simulink model "Rob_Tracking_lab"  (R2024b)
settings: Solver=FixedStepDiscrete  StartTime=0.0  StopTime=10.0  FixedStep=0.01  RelTol=1e-3  EnableMultiTasking=on
undefined symbols (not defined in the file): C_filter, DiscIntNeverNeededParam, drv, dspblkCoreblockFVToolHelper, gbox, gcbh, K_Rob_LQR, Ki, Nu, Nx, sens, T, wheel
libraries: BalRobTbx_baselib x9
settings Model: ExtModeTrigDuration=2  Creator=aboulenien  LastModifiedBy=aboulenien
settings SolverCC: AutoInsertRateTranBlk=on
settings OptimizationCC: EnhancedBackFolding=on  PassReuseOutputArgsAs=Individual arguments  ZeroExternalMemoryAtStartup=off  ZeroInternalMemoryAtStartup=off  MaxStackSize=64  OptimizeBlockOrder=speed  DifferentSizesBufferReuse=on  OptimizationCustomize=off  EfficientTunableParamExpr=on
settings DebuggingCC: ParameterTunabilityLossMsg=error
settings HardwareCC: ProdBitPerInt=16  ProdBitPerPointer=16  ProdBitPerSizeT=16  ProdBitPerPtrDiffT=16  ProdLargestAtomicFloat=None  ProdWordSize=8  ProdHWDeviceType=Atmel->AVR
settings SFSimCC: MATLABDynamicMemAlloc=off
settings RTWCC: Description=Embedded Coder  SystemTargetFile=ert.tlc  HardwareBoard=Arduino Mega 2560  TemplateMakefile=ert_default_tmf  Toolchain=Arduino AVR  BuildConfiguration=Faster Runs
settings CodeAppCC: ForceParamTrailComments=on  IgnoreCustomStorageClasses=off  OperatorAnnotations=on  SimulinkDataObjDesc=on  SFDataObjDesc=on  InsertBlockDesc=on
settings ERTTargetCC: SupportContinuousTime=on  SupportVariableSizeSignals=on  ExtModeTransport=3  ExtModeStaticAlloc=on  ExtModeAutomaticAllocSize=off  ExtModeStaticAllocSize=2048  ExtModeMexFile=ext_xcp  ExtModeIntrfLevel=Level2 - Open  InlinedParameterPlacement=Hierarchical

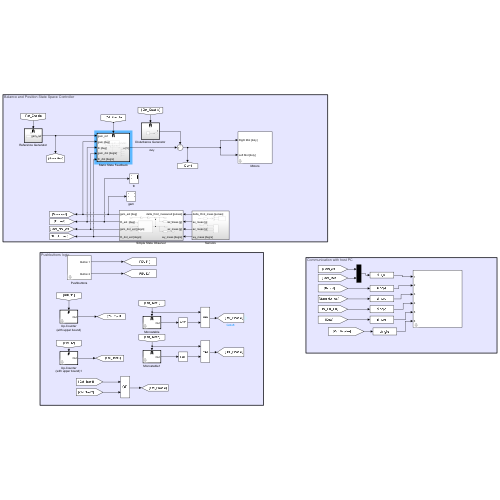
[thumbnail: Simulink's stored preview of the top-level diagram]
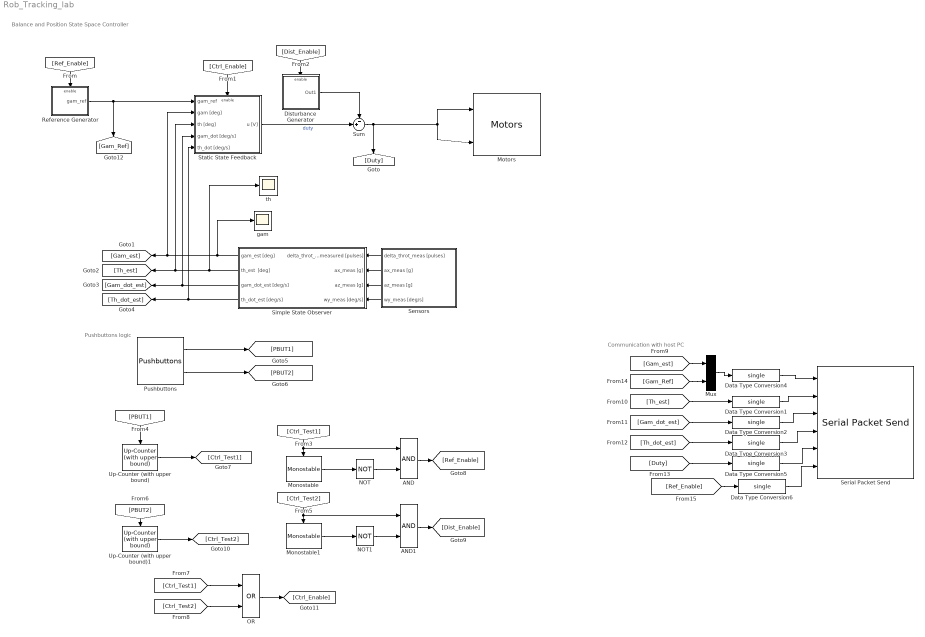
== system Rob_Tracking_lab ==
  note: Communication with host PC
  note: Balance and Position State Space Controller
  note: Pushbuttons logic
  AND : Logic  AllPortsSameDT=off  OutDataTypeStr=boolean
  AND1 : Logic  AllPortsSameDT=off  OutDataTypeStr=boolean
  Data Type Conversion{1..6} (6 alike) : DataTypeConversion  OutDataTypeStr=single  SaturateOnIntegerOverflow=off  RndMeth=Floor
  Disturbance Generator : Subsystem
  Monostable : BalRobTbx_baselib/Utilities/Monostable  Tp=5
      settings: SourceProductName=Balancing Robot Toolbox
  Monostable1 : BalRobTbx_baselib/Utilities/Monostable  Tp=1
      settings: SourceProductName=Balancing Robot Toolbox
  Motors : BalRobTbx_baselib/Outputs/Motors
      settings: SourceProductName=Balancing Robot Toolbox
  Mux : Mux  Inputs=2
  NOT : Logic  Operator=NOT  AllPortsSameDT=off  OutDataTypeStr=boolean
  NOT1 : Logic  Operator=NOT  AllPortsSameDT=off  OutDataTypeStr=boolean
  OR : Logic  Operator=OR  AllPortsSameDT=off  OutDataTypeStr=boolean
  Pushbuttons : BalRobTbx_baselib/Inputs/Pushbuttons
      settings: SourceProductName=Balancing Robot Toolbox
  Reference Generator : Subsystem
  Sensors : Subsystem
  Serial Packet Send : BalRobTbx_baselib/Communication/Serial Packet Send  serialLinkOpt=Bluetooth  baudRateOpt=38400  waitHostTxCmd=on  txStartCmd=65  txStopCmd=66  packetSpec={'2*single', 'single', 'single', 'single', 'single', 'single'}  cobsEncoded=on  nullTerminated=on  showEnablePort=off
      settings: SourceProductName=Balancing Robot Toolbox
  Simple State Observer : Subsystem
  Static State Feedback : Subsystem
  Sum : Sum  Inputs=-+|
  Up-Counter (with upper bound) : BalRobTbx_baselib/Utilities/Up-Counter (with upper bound)  CMAX=10  C0=0
      settings: SourceProductName=Balancing Robot Toolbox
  Up-Counter (with upper bound)1 : BalRobTbx_baselib/Utilities/Up-Counter (with upper bound)  CMAX=10  C0=0
      settings: SourceProductName=Balancing Robot Toolbox
  gam : Scope
  th : Scope
  wires:
  Data Type Conversion3/1 -> Serial Packet Send/4
  AND1/1 -> [Dist_Enable]
  Sensors/1(delta_throt_meas [pulses]) -> Simple State Observer/1(delta_throt_measured [pulses])
  [Ref_Enable] -> Reference Generator/Enable
  [Ctrl_Test1] -> Monostable/Enable, AND/1
  Static State Feedback/1(u [V]) -> Sum/2  "duty"
  Simple State Observer/3(gam_dot_est [deg/s]) -> Static State Feedback/4(gam_dot [deg/s]), [Gam_dot_est]
  Simple State Observer/1(gam_est [deg]) -> gam/1, Static State Feedback/2(gam [deg]), [Gam_est]
  [Ctrl_Test2] -> Monostable1/Enable, AND1/1
  [Ctrl_Test1] -> OR/1
  [Ctrl_Test2] -> OR/2
  Sensors/4(wy_meas [deg/s]) -> Simple State Observer/4(wy_meas [deg/s])
  [Ctrl_Enable] -> Static State Feedback/Enable
  Sensors/2(ax_meas [g]) -> Simple State Observer/2(ax_meas [g])
  NOT1/1 -> AND1/2
  OR/1 -> [Ctrl_Enable]
  Sensors/3(az_meas [g]) -> Simple State Observer/3(az_meas [g])
  [Dist_Enable] -> Disturbance Generator/Enable
  NOT/1 -> AND/2
  Simple State Observer/4(th_dot_est [deg/s]) -> Static State Feedback/5(th_dot [deg/s]), [Th_dot_est]
  Simple State Observer/2(th_est  [deg]) -> th/1, Static State Feedback/3(th [deg]), [Th_est]
  AND/1 -> [Ref_Enable]
  Pushbuttons/1 -> [PBUT1]
  Pushbuttons/2 -> [PBUT2]
  Data Type Conversion5/1 -> Serial Packet Send/5
  Data Type Conversion2/1 -> Serial Packet Send/3
  Data Type Conversion1/1 -> Serial Packet Send/2
  Data Type Conversion4/1 -> Serial Packet Send/1
  [Gam_est] -> Mux/1
  [Gam_Ref] -> Mux/2
  [Duty] -> Data Type Conversion5/1
  [Th_dot_est] -> Data Type Conversion3/1
  [Gam_dot_est] -> Data Type Conversion2/1
  [Th_est] -> Data Type Conversion1/1
  Mux/1 -> Data Type Conversion4/1
  Monostable1/1 -> NOT1/1
  Monostable/1 -> NOT/1
  [PBUT1] -> Up-Counter (with upper bound)/Trigger
  Up-Counter (with upper bound)/1 -> [Ctrl_Test1]
  [PBUT2] -> Up-Counter (with upper bound)1/Trigger
  Up-Counter (with upper bound)1/1 -> [Ctrl_Test2]
  [Ref_Enable] -> Data Type Conversion6/1
  Data Type Conversion6/1 -> Serial Packet Send/6
  Reference Generator/1(gam_ref) -> Static State Feedback/1(gam_ref), [Gam_Ref]
  Disturbance Generator/1(Out1) -> Sum/1
  Sum/1 -> [Duty], Motors/2, Motors/1

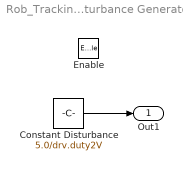
== system Rob_Tracking_lab/Disturbance Generator ==
  Enable : EnablePort  StatesWhenEnabling=reset
  Constant Disturbance : Constant  Value=5.0/drv.duty2V
  Out1 : Outport  OutputWhenDisabled=reset  InitialOutput=0
  wires:
  Constant Disturbance/1 -> Out1/1

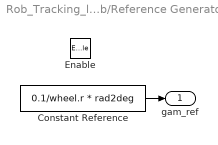
== system Rob_Tracking_lab/Reference Generator ==
  Enable : EnablePort  StatesWhenEnabling=reset
  Constant Reference : Constant  Value=0.1/wheel.r * rad2deg
  gam_ref : Outport  InitialOutput=0
  wires:
  Constant Reference/1 -> gam_ref/1

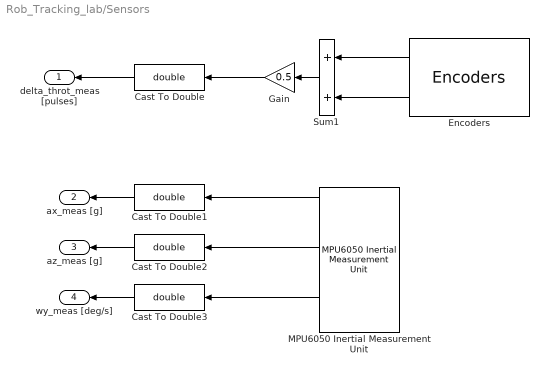
== system Rob_Tracking_lab/Sensors ==
  Cast To Double{,1..3} (4 alike) : DataTypeConversion  OutDataTypeStr=double  SaturateOnIntegerOverflow=off  RndMeth=Floor
  Encoders : BalRobTbx_baselib/Inputs/Encoders
      settings: SourceProductName=Balancing Robot Toolbox
  Gain : Gain  Gain=0.5
  MPU6050 Inertial Measurement Unit : BalRobTbx_baselib/Inputs/MPU6050 Inertial Measurement Unit
      settings: SourceProductName=Balancing Robot Toolbox
  Sum1 : Sum
  delta_throt_meas [pulses] : Outport
  ax_meas [g] : Outport  Port=2
  az_meas [g] : Outport  Port=3
  wy_meas [deg/s] : Outport  Port=4
  wires:
  Sum1/1 -> Gain/1
  Gain/1 -> Cast To Double/1
  Cast To Double/1 -> delta_throt_meas [pulses]/1
  Cast To Double3/1 -> wy_meas [deg/s]/1
  Cast To Double2/1 -> az_meas [g]/1
  Cast To Double1/1 -> ax_meas [g]/1
  Encoders/2 -> Sum1/2
  Encoders/1 -> Sum1/1
  MPU6050 Inertial Measurement Unit/1 -> Cast To Double1/1
  MPU6050 Inertial Measurement Unit/3 -> Cast To Double2/1
  MPU6050 Inertial Measurement Unit/5 -> Cast To Double3/1

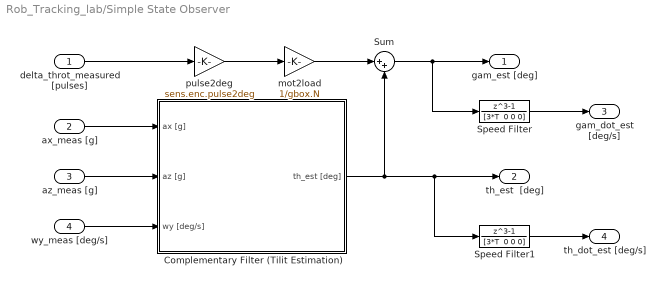
== system Rob_Tracking_lab/Simple State Observer ==
  delta_throt_measured [pulses] : Inport
  ax_meas [g] : Inport  Port=2
  az_meas [g] : Inport  Port=3
  wy_meas [deg/s] : Inport  Port=4
  Complementary Filter (Tilit Estimation) : Subsystem
  Speed Filter : DiscreteTransferFcn  LoadFcn=dspblkCoreblockFVToolHelper(gcbh,'load');  Numerator=[1 0 0 -1]  Denominator="[3*T  0 0 0]"
      settings: CopyFcn=dspblkCoreblockFVToolHelper(gcbh,'copy');  DeleteFcn=dspblkCoreblockFVToolHelper(gcbh,'close');  ModelCloseFcn=dspblkCoreblockFVToolHelper(gcbh,'close');  PreSaveFcn=dspblkCoreblockFVToolHelper(gcbh,'presave');  PostSaveFcn=dspblkCoreblockFVToolHelper(gcbh,'postsave');  CloseFcn=dspblkCoreblockFVToolHelper(gcbh,'close');
  Speed Filter1 : DiscreteTransferFcn  LoadFcn=dspblkCoreblockFVToolHelper(gcbh,'load');  Numerator=[1 0 0 -1]  Denominator="[3*T  0 0 0]"
      settings: CopyFcn=dspblkCoreblockFVToolHelper(gcbh,'copy');  DeleteFcn=dspblkCoreblockFVToolHelper(gcbh,'close');  ModelCloseFcn=dspblkCoreblockFVToolHelper(gcbh,'close');  PreSaveFcn=dspblkCoreblockFVToolHelper(gcbh,'presave');  PostSaveFcn=dspblkCoreblockFVToolHelper(gcbh,'postsave');  CloseFcn=dspblkCoreblockFVToolHelper(gcbh,'close');
  Sum : Sum  Inputs=|++
  mot2load : Gain  Gain=1/gbox.N
  pulse2deg : Gain  Gain=sens.enc.pulse2deg
  gam_est [deg] : Outport
  th_est  [deg] : Outport  Port=2
  gam_dot_est [deg/s] : Outport  Port=3
  th_dot_est [deg/s] : Outport  Port=4
  wires:
  mot2load/1 -> Sum/1
  Complementary Filter (Tilit Estimation)/1(th_est [deg]) -> th_est  [deg]/1, Speed Filter1/1, Sum/2
  Speed Filter1/1 -> th_dot_est [deg/s]/1
  delta_throt_measured [pulses]/1 -> pulse2deg/1
  Speed Filter/1 -> gam_dot_est [deg/s]/1
  pulse2deg/1 -> mot2load/1
  Sum/1 -> gam_est [deg]/1, Speed Filter/1
  ax_meas [g]/1 -> Complementary Filter (Tilit Estimation)/1(ax [g])
  az_meas [g]/1 -> Complementary Filter (Tilit Estimation)/2(az [g])
  wy_meas [deg/s]/1 -> Complementary Filter (Tilit Estimation)/3(wy [deg/s])

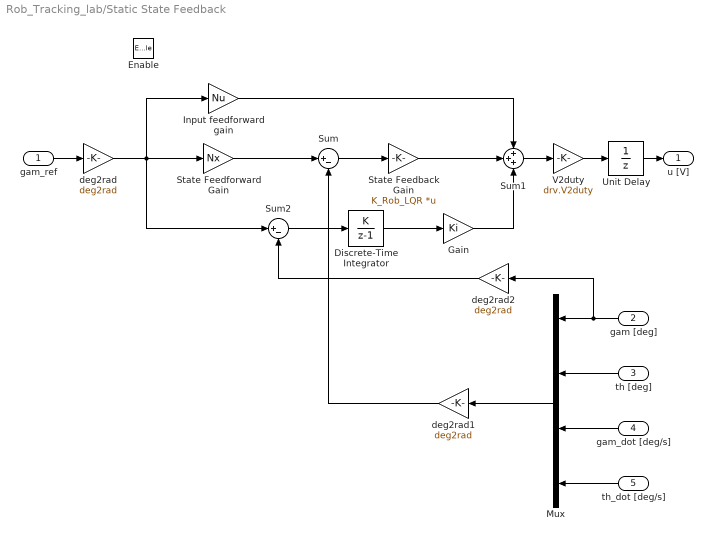
== system Rob_Tracking_lab/Static State Feedback ==
  gam_ref : Inport
  gam [deg] : Inport  Port=2
  th [deg] : Inport  Port=3
  gam_dot [deg/s] : Inport  Port=4
  th_dot [deg/s] : Inport  Port=5
  Enable : EnablePort
  Discrete-Time Integrator : DiscreteIntegrator  IntegratorMethod=Accumulation: Forward Euler  SampleTime=T  ICPrevOutput=DiscIntNeverNeededParam  ICPrevScaledInput=DiscIntNeverNeededParam
  Gain : Gain  Gain=Ki
  Input feedforward gain : Gain  Gain=Nu
  Mux : Mux
  State Feedback Gain : Gain  Gain=K_Rob_LQR  Multiplication=Matrix(K*u)
  State Feedforward Gain : Gain  Gain=Nx
  Sum : Sum  Inputs=|+-
  Sum1 : Sum  Inputs=+++
  Sum2 : Sum  Inputs=|+-
  Unit Delay : UnitDelay  SampleTime=T  HasFrameUpgradeWarning=on
  V2duty : Gain  Gain=drv.V2duty
  deg2rad : Gain  Gain=deg2rad
  deg2rad1 : Gain  Gain=deg2rad
  deg2rad2 : Gain  Gain=deg2rad
  u [V] : Outport
  wires:
  Mux/1 -> deg2rad1/1
  Discrete-Time Integrator/1 -> Gain/1
  State Feedforward Gain/1 -> Sum/1
  Unit Delay/1 -> u [V]/1
  Sum1/1 -> V2duty/1
  gam_dot [deg/s]/1 -> Mux/3
  Gain/1 -> Sum1/3
  gam_ref/1 -> deg2rad/1
  deg2rad/1 -> Sum2/1, State Feedforward Gain/1, Input feedforward gain/1
  gam [deg]/1 -> deg2rad2/1, Mux/1
  th_dot [deg/s]/1 -> Mux/4
  State Feedback Gain/1 -> Sum1/2
  deg2rad2/1 -> Sum2/2
  V2duty/1 -> Unit Delay/1
  Sum2/1 -> Discrete-Time Integrator/1
  Sum/1 -> State Feedback Gain/1
  deg2rad1/1 -> Sum/2
  Input feedforward gain/1 -> Sum1/1
  th [deg]/1 -> Mux/2

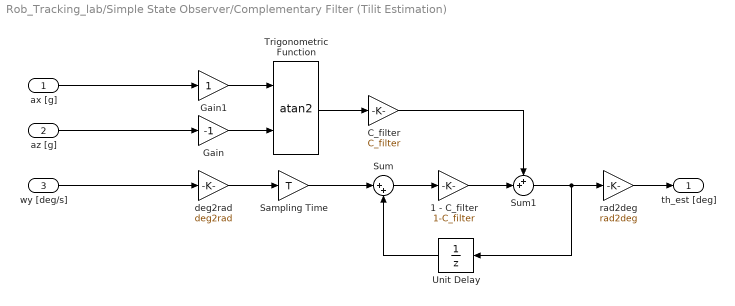
== system Rob_Tracking_lab/Simple State Observer/Complementary Filter (Tilit Estimation) ==
  ax [g] : Inport
  az [g] : Inport  Port=2
  wy [deg/s] : Inport  Port=3
  1 - C_filter : Gain  Gain=1-C_filter
  C_filter : Gain  Gain=C_filter
  Gain : Gain  Gain=-1
  Gain1 : Gain
  Sampling Time : Gain  Gain=T
  Sum : Sum  Inputs=|++
  Sum1 : Sum  Inputs=++|
  Trigonometric Function : Trigonometry  Operator=atan2
  Unit Delay : UnitDelay  SampleTime=T  HasFrameUpgradeWarning=on
  deg2rad : Gain  Gain=deg2rad
  rad2deg : Gain  Gain=rad2deg
  th_est [deg] : Outport
  wires:
  Trigonometric Function/1 -> C_filter/1
  Gain/1 -> Trigonometric Function/2
  rad2deg/1 -> th_est [deg]/1
  deg2rad/1 -> Sampling Time/1
  Sum/1 -> 1 - C_filter/1
  Gain1/1 -> Trigonometric Function/1
  Sum1/1 -> Unit Delay/1, rad2deg/1
  Sampling Time/1 -> Sum/1
  1 - C_filter/1 -> Sum1/2
  Unit Delay/1 -> Sum/2
  C_filter/1 -> Sum1/1
  ax [g]/1 -> Gain1/1
  az [g]/1 -> Gain/1
  wy [deg/s]/1 -> deg2rad/1
